simulink model "Turbine_State_Machine_Testrig"  (R2025a)
settings: Solver=ode45  StartTime=0.0  StopTime=20  MaxStep=1e-4  RelTol=1e-3  EnableMultiTasking=on
undefined symbols (not defined in the file): sigbuilder_block
libraries: Turbine_State_Machine_Lib x1
Description:
  | Copyright 2009-2025 The MathWorks, Inc. MathWorks, Inc.
settings Model: Creator=smiller  LastModifiedBy=smiller
settings SolverCC: AlgebraicLoopSolver=TrustRegion
settings DataIOCC: LimitDataPoints=on  SaveFormat=Array  SignalLoggingSaveFormat=ModelDataLogs  ReturnWorkspaceOutputs=off
settings OptimizationCC: ReuseModelBlockBuffer=off  ExpressionDepthLimit=2147483647.0  LifeSpan=inf
settings DebuggingCC: UnderspecifiedInitializationDetection=Classic  MergeDetectMultiDrivingBlocksExec=none  FcnCallInpInsideContextMsg=warning  UnconnectedInputMsg=warning  UnconnectedOutputMsg=warning  UnconnectedLineMsg=warning  AllowSymbolicDim=off  StateNameClashWarn=warning  PregeneratedLibrarySubsystemCodeDiagnostic=none  SFUnexpectedBacktrackingDiag=warning  SFNoUnconditionalDefaultTransitionDiag=warning  SFExecutionAtInitializationDiag=none  ArithmeticOperatorsInVariantConditions=warning
settings HardwareCC: ProdBitPerPointer=32.0  ProdBitPerSizeT=32.0  ProdBitPerPtrDiffT=32.0  ProdLargestAtomicFloat=None  ProdIntDivRoundTo=Undefined  ProdEndianess=Unspecified  ProdWordSize=32.0  ProdHWDeviceType=32-bit Generic
settings ModelReferenceCC: EnableRefExpFcnMdlSchedulingChecks=on  PropagateSignalLabelsOutOfModel=off
settings SFSimCC: SimUseLocalCustomCode=off  SimParseCustomCode=off  CustomCodeUndefinedFunction=UseInterfaceOnly
settings RTWCC: RTWUseLocalCustomCode=off  GPUComputeCapability=3.5  DLArmComputeVersion=19.05
settings CodeAppCC: StateflowObjectComments=on
settings GRTTargetCC: TargetLangStandard=C89/C90 (ANSI)  CombineOutputUpdateFcns=off  GRTInterface=on
settings ConfigComp: CovMetricSettings=dw  CovSaveCumulativeToWorkspaceVar=on  CovSaveSingleToWorkspaceVar=on  CovExternalEMLEnable=off  CovSFcnEnable=off

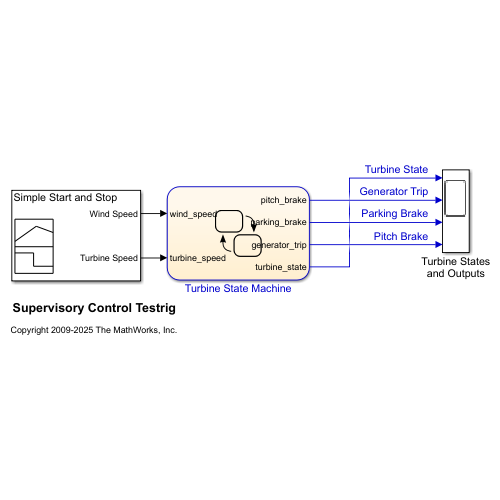
[thumbnail: Simulink's stored preview of the top-level diagram]
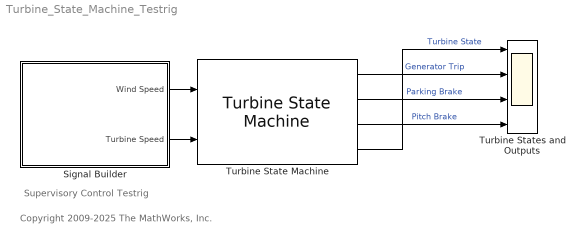
== system Turbine_State_Machine_Testrig ==
  note: Copyright 2009-2025 The MathWorks, Inc.
  note: Supervisory Control Testrig
  Signal Builder : Subsystem  Tag=STV Subsys  LoadFcn=sigbuilder_block('load');  StartFcn=sigbuilder_block('start');  StopFcn=sigbuilder_block('stop');  ClipboardFcn=sigbuilder_block('clipboard');  mask(Sigbuilder block){tuvar=[0:10]}
      mask help: Sigbuilder GUI
      mask init:
      | if ~strcmp(get_param(bdroot(gcbh),'SimulationStatus'),'stopped') tuvar = sigbuilder_block('maskInit'); end
      settings: CopyFcn=sigbuilder_block('copy');  DeleteFcn=sigbuilder_block('delete');  ModelCloseFcn=sigbuilder_block('modelClose');  PreSaveFcn=sigbuilder_block('preSave');  PauseFcn=sigbuilder_block('pause')  ContinueFcn=sigbuilder_block('continue')  NameChangeFcn=sigbuilder_block('namechange');  OpenFcn=sigbuilder_block('open',[3 32.25 762 490.5 ]);  CloseFcn=sigbuilder_block('close');
      mask Display: plot(0, 0, 100, 100,[2, 2, 32, 32, 2], [68, 8, 8, 68, 68],[32, 2], [38, 38], [32, 19, 2],[53, 60, 44], [32, 17, 17, 2],[16, 16, 31, 31]);txt = getActiveGroup(gcbh);text(2, 100, txt,'verticalAlignment', 'top');
  Turbine State Machine : Turbine_State_Machine_Lib/Turbine State Machine  SystemSampleTime=-1  VariantActivationTime=update diagram  EmptyChoice=off  PassThrough=off  PassThroughVariantControl=(default)  EmptyChoiceVariantControl=(default)  AllowFlexibleInterface=on  Latency=0  AutoFrameSizeCalculation=off
  Turbine States and Outputs : Scope  NumInputPorts=4
      settings: ActiveDisplayYMinimum=-5  ActiveDisplayYMaximum=5
  wires:
  Turbine State Machine/4 -> Turbine States and Outputs/1  "Turbine State"
  Signal Builder/1(Wind Speed) -> Turbine State Machine/1
  Signal Builder/2(Turbine Speed) -> Turbine State Machine/2
  Turbine State Machine/1 -> Turbine States and Outputs/2  "Generator Trip"
  Turbine State Machine/2 -> Turbine States and Outputs/3  "Parking Brake"
  Turbine State Machine/3 -> Turbine States and Outputs/4  "Pitch Brake"

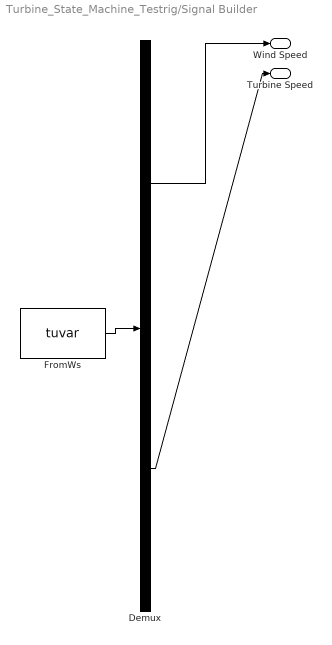
== system Turbine_State_Machine_Testrig/Signal Builder ==
  Demux : Demux  Tag=STV Demux  Outputs=2
      settings: DisplayOption=none
  FromWs : FromWorkspace  Tag=STV FromWs  VariableName=tuvar
      SigBuilderData=|
      | common.afterFinalStr = 'Extrapolate'
      | common.sampleTime = 0
      | dataSet(1).timeRange = [0 20]
      | dataSet(1).name = 'Simple Start and Stop'
      | dataSet(2).timeRange = [0 20]
      | dataSet(2).name = 'High Winds'
      | dataSet(3).timeRange = [0 20]
      | dataSet(3).name = 'Turbine Overspeed'
      | sbobj.Groups(1).Name = 'Simple Start and Stop'
      | sbobj.Groups(1).Signals(1).Name = 'Wind Speed'
      | sbobj.Groups(1).Signals(1).XData = [0 6 8.66 14 20]
      | sbobj.Groups(1).Signals(1).YData = [0 10 10 0 0]
      | sbobj.Groups(1).Signals(2).Name = 'Turbine Speed'
      | sbobj.Groups(1).Signals(2).XData = [0 4.42 4.42 6.46 10.02 16 20]
      | sbobj.Groups(1).Signals(2).YData = [0 0 0.37 1800 1800 0 0]
      | sbobj.Groups(2).Name = 'High Winds'
      | sbobj.Groups(2).Signals(1).Name = 'Wind Speed'
      | sbobj.Groups(2).Signals(1).XData = [0 4 6 8.66 20]
      | sbobj.Groups(2).Signals(1).YData = [0 10 10 22 22]
      | sbobj.Groups(2).Signals(2).Name = 'Turbine Speed'
      | sbobj.Groups(2).Signals(2).XData = [0 4.42 4.42 6.46 10.02 11.98 11.98 20]
      | sbobj.Groups(2).Signals(2).YData = [0 0 0.37 1800 1800 20 0 0]
      | sbobj.Groups(3).Name = 'Turbine Overspeed'
      | sbobj.Groups(3).Signals(1).Name = 'Wind Speed'
      | sbobj.Groups(3).Signals(1).XData = [0 4 6 8.66 14.85 20]
      | sbobj.Groups(3).Signals(1).YData = [0 10 10 12 12 12]
      | sbobj.Groups(3).Signals(2).Name = 'Turbine Speed'
      | sbobj.Groups(3).Signals(2).XData = [0 4.42 4.42 6.46 10.02 11.98 15.5 18.94 20]
      | sbobj.Groups(3).Signals(2).YData = [0 0 0.37 1800 1800 2200 2200 0 0]
  Wind Speed : Outport  Tag=STV Outport  VectorParamsAs1DForOutWhenUnconnected=off
  Turbine Speed : Outport  Tag=STV Outport  Port=2  VectorParamsAs1DForOutWhenUnconnected=off
  wires:
  Demux/1 -> Wind Speed/1
  FromWs/1 -> Demux/1
  Demux/2 -> Turbine Speed/1
